simulink model "gm_HFMA_4B_1_5_9_13"  (R2026b)
settings: Solver=FixedStepDiscrete  StopTime=stopTime  FixedStep=1.953125e-06
PreLoadFcn:
  | load('a_luts.mat')
undefined symbols (not defined in the file or in its folder): Ts
libraries: simulink x202, simulink_need_slupdate x99, hdlsllib x91
(part 16 of 20)

== system gm_HFMA_4B_1_5_9_13/Subsystem/HFMA9/crp_temp_shared4 ==
  in0 : Inport  OutDataTypeStr=fixdt(1,18,16,'DataTypeOverride', 'Off')  PortDimensions=1  SampleTime=1.953125e-06
  in1 : Inport  Port=2  OutDataTypeStr=fixdt(1,18,16,'DataTypeOverride', 'Off')  PortDimensions=1  SampleTime=1.953125e-06
  in2 : Inport  Port=3  OutDataTypeStr=fixdt(1,18,16,'DataTypeOverride', 'Off')  PortDimensions=1  SampleTime=1.953125e-06
  in3 : Inport  Port=4  OutDataTypeStr=fixdt(1,18,16,'DataTypeOverride', 'Off')  PortDimensions=1  SampleTime=1.953125e-06
  enb_counter : Inport  Port=5  OutDataTypeStr=fixdt(0,6,0,'DataTypeOverride', 'Off')  PortDimensions=1  SampleTime=1.953125e-06
  Serializer_Subnetwork : Subsystem
  Serializer_Subnetwork1 : Subsystem
  b0_2_const : Constant  Value=0.00121574103832244873046875  OutDataTypeStr=fixdt(1, 18, 26)  SampleTime=1.953125e-06
  b0_2_const1 : Constant  Value=0.00121574103832244873046875  OutDataTypeStr=fixdt(1, 18, 26)  SampleTime=1.953125e-06
  b0_2_const2 : Constant  Value=0.00121574103832244873046875  OutDataTypeStr=fixdt(1, 18, 26)  SampleTime=1.953125e-06
  b1_2 : Product  Inputs=**  OutDataTypeStr=fixdt(1, 36, 0)  SampleTime=1.953125e-06
  b1_2_const{,1..3} (4 alike) : Constant  Value=0.0024314820766448974609375  OutDataTypeStr=fixdt(1, 18, 25)  SampleTime=1.953125e-06
  b2_2_const : Constant  Value=0.00121574103832244873046875  OutDataTypeStr=fixdt(1, 18, 26)  SampleTime=1.953125e-06
  b2_2_const1 : Constant  Value=0.00121574103832244873046875  OutDataTypeStr=fixdt(1, 18, 26)  SampleTime=1.953125e-06
  b2_2_const2 : Constant  Value=0.00121574103832244873046875  OutDataTypeStr=fixdt(1, 18, 26)  SampleTime=1.953125e-06
  counter : Subsystem
  counter_matching_delay : Delay  DelayLength=80  InitialCondition=0  SampleTime=1.953125e-06
  delayMatch : Delay  DelayLength=56  InitialCondition=0  SampleTime=1.953125e-06
  delayMatch{1..13} (13 alike) : Delay  DelayLength=16  InitialCondition=0  SampleTime=1.953125e-06
  delayMatch14 : Delay  DelayLength=24  InitialCondition=0  SampleTime=1.953125e-06
  demux : Demux  Outputs=16
  enb_counter_eq_31 : simulink/Logic and Bit Operations/Compare To Constant  relop===  const=31  OutDataTypeStr=boolean
  enb_counter_ge_16 : simulink/Logic and Bit Operations/Compare To Constant  relop=>=  const=16  OutDataTypeStr=boolean
  enb_counter_ge_16_and_enb_counter_le_31 : Logic  AllPortsSameDT=off  OutDataTypeStr=boolean  SampleTime=1.953125e-06
  enb_counter_le_15 : simulink/Logic and Bit Operations/Compare To Constant  relop=<=  const=15  OutDataTypeStr=boolean
  enb_counter_le_31 : simulink/Logic and Bit Operations/Compare To Constant  relop=<=  const=31  OutDataTypeStr=boolean
  mux : Mux  Inputs=16
  mux1 : Mux  Inputs=16
  na1_1_const : Constant  Value=1.872802734375  OutDataTypeStr=fixdt(1, 18, 16)  SampleTime=1.953125e-06
  na1_1_const1 : Constant  Value=1.872802734375  OutDataTypeStr=fixdt(1, 18, 16)  SampleTime=1.953125e-06
  na1_1_const2 : Constant  Value=1.872802734375  OutDataTypeStr=fixdt(1, 18, 16)  SampleTime=1.953125e-06
  na2_1_const : Constant  Value=-0.87749481201171875  OutDataTypeStr=fixdt(1, 18, 17)  SampleTime=1.953125e-06
  na2_1_const1 : Constant  Value=-0.87749481201171875  OutDataTypeStr=fixdt(1, 18, 17)  SampleTime=1.953125e-06
  na2_1_const2 : Constant  Value=-0.87749481201171875  OutDataTypeStr=fixdt(1, 18, 17)  SampleTime=1.953125e-06
  nequ_dtc{,1..31} (32 alike) : DataTypeConversion  OutDataTypeStr=fixdt(1, 18, 0)  ConvertRealWorld=Stored Integer (SI)  SampleTime=1.953125e-06  SaturateOnIntegerOverflow=off  RndMeth=Floor
  nequ_dtc{32,37,42,47} (4 alike) : DataTypeConversion  OutDataTypeStr=fixdt(1, 36, 41)  ConvertRealWorld=Stored Integer (SI)  SampleTime=1.953125e-06  SaturateOnIntegerOverflow=off  RndMeth=Floor
  nequ_dtc33 : DataTypeConversion  OutDataTypeStr=fixdt(1, 36, 33)  ConvertRealWorld=Stored Integer (SI)  SampleTime=1.953125e-06  SaturateOnIntegerOverflow=off  RndMeth=Floor
  nequ_dtc34 : DataTypeConversion  OutDataTypeStr=fixdt(1, 36, 32)  ConvertRealWorld=Stored Integer (SI)  SampleTime=1.953125e-06  SaturateOnIntegerOverflow=off  RndMeth=Floor
  nequ_dtc{35..36,40..41,45..46} (6 alike) : DataTypeConversion  OutDataTypeStr=fixdt(1, 36, 42)  ConvertRealWorld=Stored Integer (SI)  SampleTime=1.953125e-06  SaturateOnIntegerOverflow=off  RndMeth=Floor
  nequ_dtc38 : DataTypeConversion  OutDataTypeStr=fixdt(1, 36, 33)  ConvertRealWorld=Stored Integer (SI)  SampleTime=1.953125e-06  SaturateOnIntegerOverflow=off  RndMeth=Floor
  nequ_dtc39 : DataTypeConversion  OutDataTypeStr=fixdt(1, 36, 32)  ConvertRealWorld=Stored Integer (SI)  SampleTime=1.953125e-06  SaturateOnIntegerOverflow=off  RndMeth=Floor
  nequ_dtc43 : DataTypeConversion  OutDataTypeStr=fixdt(1, 36, 33)  ConvertRealWorld=Stored Integer (SI)  SampleTime=1.953125e-06  SaturateOnIntegerOverflow=off  RndMeth=Floor
  nequ_dtc44 : DataTypeConversion  OutDataTypeStr=fixdt(1, 36, 32)  ConvertRealWorld=Stored Integer (SI)  SampleTime=1.953125e-06  SaturateOnIntegerOverflow=off  RndMeth=Floor
  tapped_delay : hdlsllib/Discrete/Tapped Delay Enabled Synchronous  vinit=0  samptime=-1  NumDelays=15  DelayOrder=Oldest  includeCurrent=on
  tapped_delay_outunit_delay : simulink_need_slupdate/Unit Delay Enabled  vinit=0.0  tsamp=-1
  out0 : Outport  OutDataTypeStr=fixdt(1,36,41,'DataTypeOverride', 'Off')  PortDimensions=1  SampleTime=1.953125e-06
  out1 : Outport  Port=2  OutDataTypeStr=fixdt(1,36,33,'DataTypeOverride', 'Off')  PortDimensions=1  SampleTime=1.953125e-06
  out2 : Outport  Port=3  OutDataTypeStr=fixdt(1,36,32,'DataTypeOverride', 'Off')  PortDimensions=1  SampleTime=1.953125e-06
  out3 : Outport  Port=4  OutDataTypeStr=fixdt(1,36,42,'DataTypeOverride', 'Off')  PortDimensions=1  SampleTime=1.953125e-06
  out4 : Outport  Port=5  OutDataTypeStr=fixdt(1,36,42,'DataTypeOverride', 'Off')  PortDimensions=1  SampleTime=1.953125e-06
  out5 : Outport  Port=6  OutDataTypeStr=fixdt(1,36,41,'DataTypeOverride', 'Off')  PortDimensions=1  SampleTime=1.953125e-06
  out6 : Outport  Port=7  OutDataTypeStr=fixdt(1,36,33,'DataTypeOverride', 'Off')  PortDimensions=1  SampleTime=1.953125e-06
  out7 : Outport  Port=8  OutDataTypeStr=fixdt(1,36,32,'DataTypeOverride', 'Off')  PortDimensions=1  SampleTime=1.953125e-06
  out8 : Outport  Port=9  OutDataTypeStr=fixdt(1,36,42,'DataTypeOverride', 'Off')  PortDimensions=1  SampleTime=1.953125e-06
  out9 : Outport  Port=10  OutDataTypeStr=fixdt(1,36,42,'DataTypeOverride', 'Off')  PortDimensions=1  SampleTime=1.953125e-06
  out10 : Outport  Port=11  OutDataTypeStr=fixdt(1,36,41,'DataTypeOverride', 'Off')  PortDimensions=1  SampleTime=1.953125e-06
  out11 : Outport  Port=12  OutDataTypeStr=fixdt(1,36,33,'DataTypeOverride', 'Off')  PortDimensions=1  SampleTime=1.953125e-06
  out12 : Outport  Port=13  OutDataTypeStr=fixdt(1,36,32,'DataTypeOverride', 'Off')  PortDimensions=1  SampleTime=1.953125e-06
  out13 : Outport  Port=14  OutDataTypeStr=fixdt(1,36,42,'DataTypeOverride', 'Off')  PortDimensions=1  SampleTime=1.953125e-06
  out14 : Outport  Port=15  OutDataTypeStr=fixdt(1,36,42,'DataTypeOverride', 'Off')  PortDimensions=1  SampleTime=1.953125e-06
  out15 : Outport  Port=16  OutDataTypeStr=fixdt(1,36,41,'DataTypeOverride', 'Off')  PortDimensions=1  SampleTime=1.953125e-06
  wires:
  nequ_dtc25/1 -> delayMatch10/1
  b1_2_const/1 -> nequ_dtc/1
  na1_1_const/1 -> nequ_dtc2/1
  nequ_dtc27/1 -> delayMatch12/1
  na2_1_const/1 -> nequ_dtc1/1
  b0_2_const1/1 -> nequ_dtc9/1
  mux1/1 -> Serializer_Subnetwork1/1(in0)
  b2_2_const/1 -> nequ_dtc3/1
  b1_2_const1/1 -> nequ_dtc5/1
  na1_1_const1/1 -> nequ_dtc7/1
  nequ_dtc15/1 -> mux/16
  b1_2_const2/1 -> nequ_dtc10/1
  b2_2_const1/1 -> nequ_dtc8/1
  b0_2_const/1 -> nequ_dtc4/1
  na2_1_const1/1 -> nequ_dtc6/1
  b1_2_const3/1 -> nequ_dtc15/1
  b2_2_const2/1 -> nequ_dtc13/1
  na2_1_const2/1 -> nequ_dtc11/1
  nequ_dtc17/1 -> delayMatch2/1
  mux/1 -> Serializer_Subnetwork/1(in0)
  b0_2_const2/1 -> nequ_dtc14/1
  na1_1_const2/1 -> nequ_dtc12/1
  delayMatch13/1 -> mux1/13
  in0/1 -> nequ_dtc18/1, nequ_dtc17/1, nequ_dtc16/1
  delayMatch7/1 -> mux1/7
  in1/1 -> nequ_dtc22/1, nequ_dtc21/1, nequ_dtc23/1, nequ_dtc20/1, nequ_dtc19/1
  delayMatch9/1 -> mux1/9
  in2/1 -> nequ_dtc28/1, nequ_dtc27/1, nequ_dtc26/1, nequ_dtc24/1, nequ_dtc25/1
  nequ_dtc18/1 -> delayMatch3/1
  enb_counter/1 -> enb_counter_le_31/1, enb_counter_ge_16/1, enb_counter_le_15/1, enb_counter_eq_31/1
  nequ_dtc36/1 -> out4/1
  nequ_dtc/1 -> mux/1
  nequ_dtc1/1 -> mux/2
  nequ_dtc2/1 -> mux/3
  nequ_dtc6/1 -> mux/7
  nequ_dtc3/1 -> mux/4
  nequ_dtc40/1 -> out8/1
  nequ_dtc4/1 -> mux/5
  nequ_dtc5/1 -> mux/6
  enb_counter_le_31/1 -> enb_counter_ge_16_and_enb_counter_le_31/2
  nequ_dtc7/1 -> mux/8
  nequ_dtc8/1 -> mux/9
  nequ_dtc13/1 -> mux/14
  nequ_dtc9/1 -> mux/10
  nequ_dtc10/1 -> mux/11
  nequ_dtc11/1 -> mux/12
  nequ_dtc12/1 -> mux/13
  nequ_dtc14/1 -> mux/15
  nequ_dtc16/1 -> delayMatch1/1
  in3/1 -> nequ_dtc30/1, nequ_dtc31/1, nequ_dtc29/1
  nequ_dtc23/1 -> delayMatch8/1
  nequ_dtc19/1 -> delayMatch4/1
  nequ_dtc20/1 -> delayMatch5/1
  nequ_dtc21/1 -> delayMatch6/1
  nequ_dtc22/1 -> delayMatch7/1
  enb_counter_le_15/1 -> counter/Enable
  nequ_dtc28/1 -> delayMatch13/1
  nequ_dtc24/1 -> delayMatch9/1
  nequ_dtc26/1 -> delayMatch11/1
  enb_counter_ge_16/1 -> enb_counter_ge_16_and_enb_counter_le_31/1
  delayMatch1/1 -> mux1/1
  delayMatch6/1 -> mux1/6
  delayMatch2/1 -> mux1/2
  delayMatch3/1 -> mux1/3
  delayMatch4/1 -> mux1/4
  delayMatch5/1 -> mux1/5
  delayMatch8/1 -> mux1/8
  counter/1(out0) -> counter_matching_delay/1, Serializer_Subnetwork/2(in1)
  delayMatch10/1 -> mux1/10
  delayMatch11/1 -> mux1/11
  delayMatch12/1 -> mux1/12
  nequ_dtc29/1 -> mux1/14
  nequ_dtc30/1 -> mux1/15
  nequ_dtc31/1 -> mux1/16
  enb_counter_ge_16_and_enb_counter_le_31/1 -> tapped_delay/2
  Serializer_Subnetwork/1(out0) -> delayMatch/1
  counter_matching_delay/1 -> Serializer_Subnetwork1/2(in1)
  delayMatch/1 -> delayMatch14/1
  Serializer_Subnetwork1/1(out0) -> b1_2/2
  delayMatch14/1 -> b1_2/1
  enb_counter_eq_31/1 -> tapped_delay_outunit_delay/2
  b1_2/1 -> tapped_delay/1
  tapped_delay/1 -> tapped_delay_outunit_delay/1
  tapped_delay_outunit_delay/1 -> demux/1
  demux/1 -> nequ_dtc32/1
  demux/2 -> nequ_dtc33/1
  demux/3 -> nequ_dtc34/1
  demux/4 -> nequ_dtc35/1
  demux/5 -> nequ_dtc36/1
  demux/6 -> nequ_dtc37/1
  demux/7 -> nequ_dtc38/1
  demux/8 -> nequ_dtc39/1
  demux/9 -> nequ_dtc40/1
  demux/10 -> nequ_dtc41/1
  demux/11 -> nequ_dtc42/1
  demux/12 -> nequ_dtc43/1
  demux/13 -> nequ_dtc44/1
  demux/14 -> nequ_dtc45/1
  demux/15 -> nequ_dtc46/1
  demux/16 -> nequ_dtc47/1
  nequ_dtc32/1 -> out0/1
  nequ_dtc33/1 -> out1/1
  nequ_dtc34/1 -> out2/1
  nequ_dtc35/1 -> out3/1
  nequ_dtc37/1 -> out5/1
  nequ_dtc38/1 -> out6/1
  nequ_dtc39/1 -> out7/1
  nequ_dtc41/1 -> out9/1
  nequ_dtc42/1 -> out10/1
  nequ_dtc43/1 -> out11/1
  nequ_dtc44/1 -> out12/1
  nequ_dtc45/1 -> out13/1
  nequ_dtc46/1 -> out14/1
  nequ_dtc47/1 -> out15/1

== system gm_HFMA_4B_1_5_9_13/Subsystem/HFMA9/crp_temp_shared5 ==
  in0 : Inport  OutDataTypeStr=fixdt(1,18,16,'DataTypeOverride', 'Off')  PortDimensions=1  SampleTime=1.953125e-06
  in1 : Inport  Port=2  OutDataTypeStr=fixdt(1,18,16,'DataTypeOverride', 'Off')  PortDimensions=1  SampleTime=1.953125e-06
  in2 : Inport  Port=3  OutDataTypeStr=fixdt(1,18,16,'DataTypeOverride', 'Off')  PortDimensions=1  SampleTime=1.953125e-06
  in3 : Inport  Port=4  OutDataTypeStr=fixdt(1,18,16,'DataTypeOverride', 'Off')  PortDimensions=1  SampleTime=1.953125e-06
  enb_counter : Inport  Port=5  OutDataTypeStr=fixdt(0,6,0,'DataTypeOverride', 'Off')  PortDimensions=1  SampleTime=1.953125e-06
  Serializer_Subnetwork : Subsystem
  Serializer_Subnetwork1 : Subsystem
  b0_2_const : Constant  Value=0.00121574103832244873046875  OutDataTypeStr=fixdt(1, 18, 26)  SampleTime=1.953125e-06
  b0_2_const1 : Constant  Value=0.00121574103832244873046875  OutDataTypeStr=fixdt(1, 18, 26)  SampleTime=1.953125e-06
  b0_2_const2 : Constant  Value=0.00121574103832244873046875  OutDataTypeStr=fixdt(1, 18, 26)  SampleTime=1.953125e-06
  b1_2_const : Constant  Value=0.0024314820766448974609375  OutDataTypeStr=fixdt(1, 18, 25)  SampleTime=1.953125e-06
  b1_2_const1 : Constant  Value=0.0024314820766448974609375  OutDataTypeStr=fixdt(1, 18, 25)  SampleTime=1.953125e-06
  b1_2_const2 : Constant  Value=0.0024314820766448974609375  OutDataTypeStr=fixdt(1, 18, 25)  SampleTime=1.953125e-06
  b2_2_const : Constant  Value=0.00121574103832244873046875  OutDataTypeStr=fixdt(1, 18, 26)  SampleTime=1.953125e-06
  b2_2_const1 : Constant  Value=0.00121574103832244873046875  OutDataTypeStr=fixdt(1, 18, 26)  SampleTime=1.953125e-06
  b2_2_const2 : Constant  Value=0.00121574103832244873046875  OutDataTypeStr=fixdt(1, 18, 26)  SampleTime=1.953125e-06
  counter : Subsystem
  counter_matching_delay : Delay  DelayLength=80  InitialCondition=0  SampleTime=1.953125e-06
  delayMatch : Delay  DelayLength=56  InitialCondition=0  SampleTime=1.953125e-06
  delayMatch1 : Delay  DelayLength=24  InitialCondition=0  SampleTime=1.953125e-06
  demux : Demux  Outputs=16
  enb_counter_eq_31 : simulink/Logic and Bit Operations/Compare To Constant  relop===  const=31  OutDataTypeStr=boolean
  enb_counter_ge_16 : simulink/Logic and Bit Operations/Compare To Constant  relop=>=  const=16  OutDataTypeStr=boolean
  enb_counter_ge_16_and_enb_counter_le_31 : Logic  AllPortsSameDT=off  OutDataTypeStr=boolean  SampleTime=1.953125e-06
  enb_counter_le_15 : simulink/Logic and Bit Operations/Compare To Constant  relop=<=  const=15  OutDataTypeStr=boolean
  enb_counter_le_31 : simulink/Logic and Bit Operations/Compare To Constant  relop=<=  const=31  OutDataTypeStr=boolean
  mux : Mux  Inputs=16
  mux1 : Mux  Inputs=16
  na1_1_const : Constant  Value=1.872802734375  OutDataTypeStr=fixdt(1, 18, 16)  SampleTime=1.953125e-06
  na1_1_const1 : Constant  Value=1.872802734375  OutDataTypeStr=fixdt(1, 18, 16)  SampleTime=1.953125e-06
  na1_1_const2 : Constant  Value=1.872802734375  OutDataTypeStr=fixdt(1, 18, 16)  SampleTime=1.953125e-06
  na2_1 : Product  Inputs=**  OutDataTypeStr=fixdt(1, 36, 0)  SampleTime=1.953125e-06
  na2_1_const{,1..3} (4 alike) : Constant  Value=-0.87749481201171875  OutDataTypeStr=fixdt(1, 18, 17)  SampleTime=1.953125e-06
  nequ_dtc{,1..31} (32 alike) : DataTypeConversion  OutDataTypeStr=fixdt(1, 18, 0)  ConvertRealWorld=Stored Integer (SI)  SampleTime=1.953125e-06  SaturateOnIntegerOverflow=off  RndMeth=Floor
  nequ_dtc{32,37,42,47} (4 alike) : DataTypeConversion  OutDataTypeStr=fixdt(1, 36, 33)  ConvertRealWorld=Stored Integer (SI)  SampleTime=1.953125e-06  SaturateOnIntegerOverflow=off  RndMeth=Floor
  nequ_dtc33 : DataTypeConversion  OutDataTypeStr=fixdt(1, 36, 32)  ConvertRealWorld=Stored Integer (SI)  SampleTime=1.953125e-06  SaturateOnIntegerOverflow=off  RndMeth=Floor
  nequ_dtc{34..35,39..40,44..45} (6 alike) : DataTypeConversion  OutDataTypeStr=fixdt(1, 36, 42)  ConvertRealWorld=Stored Integer (SI)  SampleTime=1.953125e-06  SaturateOnIntegerOverflow=off  RndMeth=Floor
  nequ_dtc36 : DataTypeConversion  OutDataTypeStr=fixdt(1, 36, 41)  ConvertRealWorld=Stored Integer (SI)  SampleTime=1.953125e-06  SaturateOnIntegerOverflow=off  RndMeth=Floor
  nequ_dtc38 : DataTypeConversion  OutDataTypeStr=fixdt(1, 36, 32)  ConvertRealWorld=Stored Integer (SI)  SampleTime=1.953125e-06  SaturateOnIntegerOverflow=off  RndMeth=Floor
  nequ_dtc41 : DataTypeConversion  OutDataTypeStr=fixdt(1, 36, 41)  ConvertRealWorld=Stored Integer (SI)  SampleTime=1.953125e-06  SaturateOnIntegerOverflow=off  RndMeth=Floor
  nequ_dtc43 : DataTypeConversion  OutDataTypeStr=fixdt(1, 36, 32)  ConvertRealWorld=Stored Integer (SI)  SampleTime=1.953125e-06  SaturateOnIntegerOverflow=off  RndMeth=Floor
  nequ_dtc46 : DataTypeConversion  OutDataTypeStr=fixdt(1, 36, 41)  ConvertRealWorld=Stored Integer (SI)  SampleTime=1.953125e-06  SaturateOnIntegerOverflow=off  RndMeth=Floor
  tapped_delay : hdlsllib/Discrete/Tapped Delay Enabled Synchronous  vinit=0  samptime=-1  NumDelays=15  DelayOrder=Oldest  includeCurrent=on
  tapped_delay_outunit_delay : simulink_need_slupdate/Unit Delay Enabled  vinit=0.0  tsamp=-1
  out0 : Outport  OutDataTypeStr=fixdt(1,36,33,'DataTypeOverride', 'Off')  PortDimensions=1  SampleTime=1.953125e-06
  out1 : Outport  Port=2  OutDataTypeStr=fixdt(1,36,32,'DataTypeOverride', 'Off')  PortDimensions=1  SampleTime=1.953125e-06
  out2 : Outport  Port=3  OutDataTypeStr=fixdt(1,36,42,'DataTypeOverride', 'Off')  PortDimensions=1  SampleTime=1.953125e-06
  out3 : Outport  Port=4  OutDataTypeStr=fixdt(1,36,42,'DataTypeOverride', 'Off')  PortDimensions=1  SampleTime=1.953125e-06
  out4 : Outport  Port=5  OutDataTypeStr=fixdt(1,36,41,'DataTypeOverride', 'Off')  PortDimensions=1  SampleTime=1.953125e-06
  out5 : Outport  Port=6  OutDataTypeStr=fixdt(1,36,33,'DataTypeOverride', 'Off')  PortDimensions=1  SampleTime=1.953125e-06
  out6 : Outport  Port=7  OutDataTypeStr=fixdt(1,36,32,'DataTypeOverride', 'Off')  PortDimensions=1  SampleTime=1.953125e-06
  out7 : Outport  Port=8  OutDataTypeStr=fixdt(1,36,42,'DataTypeOverride', 'Off')  PortDimensions=1  SampleTime=1.953125e-06
  out8 : Outport  Port=9  OutDataTypeStr=fixdt(1,36,42,'DataTypeOverride', 'Off')  PortDimensions=1  SampleTime=1.953125e-06
  out9 : Outport  Port=10  OutDataTypeStr=fixdt(1,36,41,'DataTypeOverride', 'Off')  PortDimensions=1  SampleTime=1.953125e-06
  out10 : Outport  Port=11  OutDataTypeStr=fixdt(1,36,33,'DataTypeOverride', 'Off')  PortDimensions=1  SampleTime=1.953125e-06
  out11 : Outport  Port=12  OutDataTypeStr=fixdt(1,36,32,'DataTypeOverride', 'Off')  PortDimensions=1  SampleTime=1.953125e-06
  out12 : Outport  Port=13  OutDataTypeStr=fixdt(1,36,42,'DataTypeOverride', 'Off')  PortDimensions=1  SampleTime=1.953125e-06
  out13 : Outport  Port=14  OutDataTypeStr=fixdt(1,36,42,'DataTypeOverride', 'Off')  PortDimensions=1  SampleTime=1.953125e-06
  out14 : Outport  Port=15  OutDataTypeStr=fixdt(1,36,41,'DataTypeOverride', 'Off')  PortDimensions=1  SampleTime=1.953125e-06
  out15 : Outport  Port=16  OutDataTypeStr=fixdt(1,36,33,'DataTypeOverride', 'Off')  PortDimensions=1  SampleTime=1.953125e-06
  wires:
  b0_2_const/1 -> nequ_dtc3/1
  nequ_dtc29/1 -> mux1/14
  na1_1_const/1 -> nequ_dtc1/1
  nequ_dtc25/1 -> mux1/10
  nequ_dtc27/1 -> mux1/12
  na2_1_const/1 -> nequ_dtc/1
  b2_2_const/1 -> nequ_dtc2/1
  demux/8 -> nequ_dtc39/1
  na1_1_const2/1 -> nequ_dtc11/1
  b1_2_const1/1 -> nequ_dtc9/1
  demux/4 -> nequ_dtc35/1
  na2_1_const1/1 -> nequ_dtc5/1
  b2_2_const1/1 -> nequ_dtc7/1
  b0_2_const1/1 -> nequ_dtc8/1
  nequ_dtc31/1 -> mux1/16
  demux/10 -> nequ_dtc41/1
  na2_1_const2/1 -> nequ_dtc10/1
  demux/6 -> nequ_dtc37/1
  b1_2_const/1 -> nequ_dtc4/1
  na1_1_const1/1 -> nequ_dtc6/1
  mux/1 -> Serializer_Subnetwork/1(in0)
  nequ_dtc19/1 -> mux1/4
  b1_2_const2/1 -> nequ_dtc14/1
  b2_2_const2/1 -> nequ_dtc12/1
  b0_2_const2/1 -> nequ_dtc13/1
  nequ_dtc17/1 -> mux1/2
  na2_1_const3/1 -> nequ_dtc15/1
  enb_counter/1 -> enb_counter_le_31/1, enb_counter_ge_16/1, enb_counter_eq_31/1, enb_counter_le_15/1
  nequ_dtc24/1 -> mux1/9
  nequ_dtc20/1 -> mux1/5
  nequ_dtc/1 -> mux/1
  nequ_dtc21/1 -> mux1/6
  nequ_dtc1/1 -> mux/2
  nequ_dtc2/1 -> mux/3
  nequ_dtc3/1 -> mux/4
  nequ_dtc42/1 -> out10/1
  nequ_dtc4/1 -> mux/5
  nequ_dtc5/1 -> mux/6
  nequ_dtc6/1 -> mux/7
  nequ_dtc7/1 -> mux/8
  nequ_dtc8/1 -> mux/9
  Serializer_Subnetwork1/1(out0) -> na2_1/2
  nequ_dtc9/1 -> mux/10
  in2/1 -> nequ_dtc25/1, nequ_dtc26/1, nequ_dtc23/1, nequ_dtc24/1, nequ_dtc27/1
  nequ_dtc14/1 -> mux/15
  nequ_dtc10/1 -> mux/11
  in3/1 -> nequ_dtc31/1, nequ_dtc30/1, nequ_dtc29/1, nequ_dtc28/1
  nequ_dtc11/1 -> mux/12
  in0/1 -> nequ_dtc17/1, nequ_dtc16/1
  nequ_dtc12/1 -> mux/13
  in1/1 -> nequ_dtc21/1, nequ_dtc20/1, nequ_dtc19/1, nequ_dtc18/1, nequ_dtc22/1
  nequ_dtc13/1 -> mux/14
  nequ_dtc15/1 -> mux/16
  enb_counter_le_15/1 -> counter/Enable
  enb_counter_ge_16/1 -> enb_counter_ge_16_and_enb_counter_le_31/1
  enb_counter_le_31/1 -> enb_counter_ge_16_and_enb_counter_le_31/2
  nequ_dtc16/1 -> mux1/1
  nequ_dtc18/1 -> mux1/3
  nequ_dtc22/1 -> mux1/7
  nequ_dtc23/1 -> mux1/8
  counter/1(out0) -> Serializer_Subnetwork/2(in1), counter_matching_delay/1
  nequ_dtc30/1 -> mux1/15
  nequ_dtc26/1 -> mux1/11
  nequ_dtc28/1 -> mux1/13
  enb_counter_ge_16_and_enb_counter_le_31/1 -> tapped_delay/2
  Serializer_Subnetwork/1(out0) -> delayMatch/1
  mux1/1 -> Serializer_Subnetwork1/1(in0)
  counter_matching_delay/1 -> Serializer_Subnetwork1/2(in1)
  delayMatch/1 -> delayMatch1/1
  delayMatch1/1 -> na2_1/1
  enb_counter_eq_31/1 -> tapped_delay_outunit_delay/2
  na2_1/1 -> tapped_delay/1
  tapped_delay/1 -> tapped_delay_outunit_delay/1
  tapped_delay_outunit_delay/1 -> demux/1
  demux/1 -> nequ_dtc32/1
  demux/2 -> nequ_dtc33/1
  demux/3 -> nequ_dtc34/1
  demux/5 -> nequ_dtc36/1
  demux/7 -> nequ_dtc38/1
  demux/9 -> nequ_dtc40/1
  demux/11 -> nequ_dtc42/1
  demux/12 -> nequ_dtc43/1
  demux/13 -> nequ_dtc44/1
  demux/14 -> nequ_dtc45/1
  demux/15 -> nequ_dtc46/1
  demux/16 -> nequ_dtc47/1
  nequ_dtc32/1 -> out0/1
  nequ_dtc33/1 -> out1/1
  nequ_dtc34/1 -> out2/1
  nequ_dtc35/1 -> out3/1
  nequ_dtc36/1 -> out4/1
  nequ_dtc37/1 -> out5/1
  nequ_dtc38/1 -> out6/1
  nequ_dtc39/1 -> out7/1
  nequ_dtc40/1 -> out8/1
  nequ_dtc41/1 -> out9/1
  nequ_dtc43/1 -> out11/1
  nequ_dtc44/1 -> out12/1
  nequ_dtc45/1 -> out13/1
  nequ_dtc46/1 -> out14/1
  nequ_dtc47/1 -> out15/1

== system gm_HFMA_4B_1_5_9_13/Subsystem/HFMA9/crp_temp_shared6 ==
  in0 : Inport  OutDataTypeStr=fixdt(1,18,16,'DataTypeOverride', 'Off')  PortDimensions=1  SampleTime=1.953125e-06
  in1 : Inport  Port=2  OutDataTypeStr=fixdt(1,18,16,'DataTypeOverride', 'Off')  PortDimensions=1  SampleTime=1.953125e-06
  in2 : Inport  Port=3  OutDataTypeStr=fixdt(1,18,16,'DataTypeOverride', 'Off')  PortDimensions=1  SampleTime=1.953125e-06
  in3 : Inport  Port=4  OutDataTypeStr=fixdt(1,18,16,'DataTypeOverride', 'Off')  PortDimensions=1  SampleTime=1.953125e-06
  in4 : Inport  Port=5  OutDataTypeStr=fixdt(1,18,16,'DataTypeOverride', 'Off')  PortDimensions=1  SampleTime=1.953125e-06
  in5 : Inport  Port=6  OutDataTypeStr=fixdt(1,18,16,'DataTypeOverride', 'Off')  PortDimensions=1  SampleTime=1.953125e-06
  in6 : Inport  Port=7  OutDataTypeStr=fixdt(1,18,16,'DataTypeOverride', 'Off')  PortDimensions=1  SampleTime=1.953125e-06
  enb_counter : Inport  Port=8  OutDataTypeStr=fixdt(0,6,0,'DataTypeOverride', 'Off')  PortDimensions=1  SampleTime=1.953125e-06
  Serializer_Subnetwork : Subsystem
  Serializer_Subnetwork1 : Subsystem
  b0_2_const : Constant  Value=0.00121574103832244873046875  OutDataTypeStr=fixdt(1, 18, 26)  SampleTime=1.953125e-06
  b1_2_const : Constant  Value=0.0024314820766448974609375  OutDataTypeStr=fixdt(1, 18, 25)  SampleTime=1.953125e-06
  b2_2_const : Constant  Value=0.00121574103832244873046875  OutDataTypeStr=fixdt(1, 18, 26)  SampleTime=1.953125e-06
  counter : Subsystem
  delayMatch{,1..7,9..12} (12 alike) : Delay  DelayLength=24  InitialCondition=0  SampleTime=1.953125e-06
  delayMatch{8,13..20} (9 alike) : Delay  DelayLength=16  InitialCondition=0  SampleTime=1.953125e-06
  demux : Demux  Outputs=16
  enb_counter_eq_47 : simulink/Logic and Bit Operations/Compare To Constant  relop===  const=47  OutDataTypeStr=boolean
  enb_counter_ge_32 : simulink/Logic and Bit Operations/Compare To Constant  relop=>=  const=32  OutDataTypeStr=boolean
  enb_counter_ge_32_and_enb_counter_le_47 : Logic  AllPortsSameDT=off  OutDataTypeStr=boolean  SampleTime=1.953125e-06
  enb_counter_le_47 : simulink/Logic and Bit Operations/Compare To Constant  relop=<=  const=47  OutDataTypeStr=boolean
  mux : Mux  Inputs=16
  mux1 : Mux  Inputs=16
  na1_1 : Product  Inputs=**  OutDataTypeStr=fixdt(1, 36, 0)  SampleTime=1.953125e-06
  na1_1_const : Constant  Value=1.872802734375  OutDataTypeStr=fixdt(1, 18, 16)  SampleTime=1.953125e-06
  na1_1_const1 : Constant  Value=1.872802734375  OutDataTypeStr=fixdt(1, 18, 16)  SampleTime=1.953125e-06
  na1_2_const : Constant  Value=1.9425048828125  OutDataTypeStr=fixdt(1, 18, 16)  SampleTime=1.953125e-06
  na1_2_const1 : Constant  Value=1.9425048828125  OutDataTypeStr=fixdt(1, 18, 16)  SampleTime=1.953125e-06
  na1_2_const2 : Constant  Value=1.9425048828125  OutDataTypeStr=fixdt(1, 18, 16)  SampleTime=1.953125e-06
  na2_1_const : Constant  Value=-0.87749481201171875  OutDataTypeStr=fixdt(1, 18, 17)  SampleTime=1.953125e-06
  na2_2_const : Constant  Value=-0.94736480712890625  OutDataTypeStr=fixdt(1, 18, 17)  SampleTime=1.953125e-06
  na2_2_const1 : Constant  Value=-0.94736480712890625  OutDataTypeStr=fixdt(1, 18, 17)  SampleTime=1.953125e-06
  na2_2_const2 : Constant  Value=-0.94736480712890625  OutDataTypeStr=fixdt(1, 18, 17)  SampleTime=1.953125e-06
  nequ_dtc{,1..31} (32 alike) : DataTypeConversion  OutDataTypeStr=fixdt(1, 18, 0)  ConvertRealWorld=Stored Integer (SI)  SampleTime=1.953125e-06  SaturateOnIntegerOverflow=off  RndMeth=Floor
  nequ_dtc{32,37,39..40,42..44,46..47} (9 alike) : DataTypeConversion  OutDataTypeStr=fixdt(1, 36, 32)  ConvertRealWorld=Stored Integer (SI)  SampleTime=1.953125e-06  SaturateOnIntegerOverflow=off  RndMeth=Floor
  nequ_dtc33 : DataTypeConversion  OutDataTypeStr=fixdt(1, 36, 42)  ConvertRealWorld=Stored Integer (SI)  SampleTime=1.953125e-06  SaturateOnIntegerOverflow=off  RndMeth=Floor
  nequ_dtc34 : DataTypeConversion  OutDataTypeStr=fixdt(1, 36, 42)  ConvertRealWorld=Stored Integer (SI)  SampleTime=1.953125e-06  SaturateOnIntegerOverflow=off  RndMeth=Floor
  nequ_dtc35 : DataTypeConversion  OutDataTypeStr=fixdt(1, 36, 41)  ConvertRealWorld=Stored Integer (SI)  SampleTime=1.953125e-06  SaturateOnIntegerOverflow=off  RndMeth=Floor
  nequ_dtc{36,38,41,45} (4 alike) : DataTypeConversion  OutDataTypeStr=fixdt(1, 36, 33)  ConvertRealWorld=Stored Integer (SI)  SampleTime=1.953125e-06  SaturateOnIntegerOverflow=off  RndMeth=Floor
  tapped_delay : hdlsllib/Discrete/Tapped Delay Enabled Synchronous  vinit=0  samptime=-1  NumDelays=15  DelayOrder=Oldest  includeCurrent=on
  tapped_delay_outunit_delay : simulink_need_slupdate/Unit Delay Enabled  vinit=0.0  tsamp=-1
  out0 : Outport  OutDataTypeStr=fixdt(1,36,32,'DataTypeOverride', 'Off')  PortDimensions=1  SampleTime=1.953125e-06
  out1 : Outport  Port=2  OutDataTypeStr=fixdt(1,36,42,'DataTypeOverride', 'Off')  PortDimensions=1  SampleTime=1.953125e-06
  out2 : Outport  Port=3  OutDataTypeStr=fixdt(1,36,42,'DataTypeOverride', 'Off')  PortDimensions=1  SampleTime=1.953125e-06
  out3 : Outport  Port=4  OutDataTypeStr=fixdt(1,36,41,'DataTypeOverride', 'Off')  PortDimensions=1  SampleTime=1.953125e-06
  out4 : Outport  Port=5  OutDataTypeStr=fixdt(1,36,33,'DataTypeOverride', 'Off')  PortDimensions=1  SampleTime=1.953125e-06
  out5 : Outport  Port=6  OutDataTypeStr=fixdt(1,36,32,'DataTypeOverride', 'Off')  PortDimensions=1  SampleTime=1.953125e-06
  out6 : Outport  Port=7  OutDataTypeStr=fixdt(1,36,33,'DataTypeOverride', 'Off')  PortDimensions=1  SampleTime=1.953125e-06
  out7 : Outport  Port=8  OutDataTypeStr=fixdt(1,36,32,'DataTypeOverride', 'Off')  PortDimensions=1  SampleTime=1.953125e-06
  out8 : Outport  Port=9  OutDataTypeStr=fixdt(1,36,32,'DataTypeOverride', 'Off')  PortDimensions=1  SampleTime=1.953125e-06
  out9 : Outport  Port=10  OutDataTypeStr=fixdt(1,36,33,'DataTypeOverride', 'Off')  PortDimensions=1  SampleTime=1.953125e-06
  out10 : Outport  Port=11  OutDataTypeStr=fixdt(1,36,32,'DataTypeOverride', 'Off')  PortDimensions=1  SampleTime=1.953125e-06
  out11 : Outport  Port=12  OutDataTypeStr=fixdt(1,36,32,'DataTypeOverride', 'Off')  PortDimensions=1  SampleTime=1.953125e-06
  out12 : Outport  Port=13  OutDataTypeStr=fixdt(1,36,32,'DataTypeOverride', 'Off')  PortDimensions=1  SampleTime=1.953125e-06
  out13 : Outport  Port=14  OutDataTypeStr=fixdt(1,36,33,'DataTypeOverride', 'Off')  PortDimensions=1  SampleTime=1.953125e-06
  out14 : Outport  Port=15  OutDataTypeStr=fixdt(1,36,32,'DataTypeOverride', 'Off')  PortDimensions=1  SampleTime=1.953125e-06
  out15 : Outport  Port=16  OutDataTypeStr=fixdt(1,36,32,'DataTypeOverride', 'Off')  PortDimensions=1  SampleTime=1.953125e-06
  wires:
  na1_1_const/1 -> nequ_dtc/1
  demux/3 -> nequ_dtc34/1
  b0_2_const/1 -> nequ_dtc2/1
  demux/15 -> nequ_dtc46/1
  na2_1_const/1 -> nequ_dtc4/1
  demux/5 -> nequ_dtc36/1
  b2_2_const/1 -> nequ_dtc1/1
  b1_2_const/1 -> nequ_dtc3/1
  na1_1_const1/1 -> nequ_dtc5/1
  nequ_dtc20/1 -> delayMatch17/1
  na1_2_const2/1 -> nequ_dtc14/1
  na1_2_const1/1 -> nequ_dtc10/1
  na1_2_const/1 -> nequ_dtc7/1
  nequ_dtc18/1 -> delayMatch15/1
  na2_2_const2/1 -> nequ_dtc13/1
  na2_2_const1/1 -> nequ_dtc9/1
  na2_2_const/1 -> nequ_dtc6/1
  in0/1 -> nequ_dtc16/1
  nequ_dtc12/1 -> mux/13
  in6/1 -> nequ_dtc15/1
  nequ_dtc16/1 -> delayMatch13/1
  in2/1 -> nequ_dtc23/1, nequ_dtc22/1, nequ_dtc8/1
  nequ_dtc13/1 -> delayMatch11/1
  in1/1 -> nequ_dtc21/1, nequ_dtc20/1, nequ_dtc19/1, nequ_dtc18/1, nequ_dtc17/1
  in3/1 -> nequ_dtc31/1, nequ_dtc29/1, nequ_dtc27/1, nequ_dtc30/1, nequ_dtc24/1
  enb_counter/1 -> enb_counter_eq_47/1, enb_counter_le_47/1, enb_counter_ge_32/1
  nequ_dtc/1 -> delayMatch/1
  nequ_dtc1/1 -> delayMatch1/1
  enb_counter_le_47/1 -> enb_counter_ge_32_and_enb_counter_le_47/2
  nequ_dtc6/1 -> delayMatch6/1
  nequ_dtc2/1 -> delayMatch2/1
  nequ_dtc3/1 -> delayMatch3/1
  nequ_dtc4/1 -> delayMatch4/1
  nequ_dtc5/1 -> delayMatch5/1
  nequ_dtc11/1 -> mux/12
  nequ_dtc7/1 -> delayMatch7/1
  nequ_dtc8/1 -> delayMatch8/1
  nequ_dtc9/1 -> delayMatch9/1
  nequ_dtc10/1 -> delayMatch10/1
  nequ_dtc14/1 -> delayMatch12/1
  nequ_dtc21/1 -> delayMatch18/1
  nequ_dtc17/1 -> delayMatch14/1
  in4/1 -> nequ_dtc26/1, nequ_dtc25/1, nequ_dtc12/1, nequ_dtc11/1
  nequ_dtc19/1 -> delayMatch16/1
  nequ_dtc22/1 -> delayMatch19/1
  nequ_dtc23/1 -> delayMatch20/1
  in5/1 -> nequ_dtc28/1
  enb_counter_ge_32/1 -> enb_counter_ge_32_and_enb_counter_le_47/1
  delayMatch4/1 -> mux/5
  delayMatch/1 -> mux/1
  delayMatch5/1 -> mux/6
  delayMatch1/1 -> mux/2
  delayMatch2/1 -> mux/3
  delayMatch3/1 -> mux/4
  delayMatch10/1 -> mux/11
  delayMatch6/1 -> mux/7
  delayMatch7/1 -> mux/8
  delayMatch8/1 -> mux/9
  delayMatch9/1 -> mux/10
  delayMatch15/1 -> mux1/3
  delayMatch11/1 -> mux/14
  delayMatch12/1 -> mux/15
  nequ_dtc15/1 -> mux/16
  delayMatch13/1 -> mux1/1
  delayMatch14/1 -> mux1/2
  delayMatch16/1 -> mux1/4
  delayMatch17/1 -> mux1/5
  delayMatch18/1 -> mux1/6
  delayMatch19/1 -> mux1/7
  delayMatch20/1 -> mux1/8
  nequ_dtc24/1 -> mux1/9
  nequ_dtc25/1 -> mux1/10
  nequ_dtc26/1 -> mux1/11
  nequ_dtc27/1 -> mux1/12
  nequ_dtc28/1 -> mux1/13
  nequ_dtc29/1 -> mux1/14
  nequ_dtc30/1 -> mux1/15
  nequ_dtc31/1 -> mux1/16
  enb_counter_ge_32_and_enb_counter_le_47/1 -> counter/Enable, tapped_delay/2
  mux/1 -> Serializer_Subnetwork/1(in0)
  mux1/1 -> Serializer_Subnetwork1/1(in0)
  counter/1(out0) -> Serializer_Subnetwork1/2(in1), Serializer_Subnetwork/2(in1)
  Serializer_Subnetwork/1(out0) -> na1_1/1
  Serializer_Subnetwork1/1(out0) -> na1_1/2
  na1_1/1 -> tapped_delay/1
  enb_counter_eq_47/1 -> tapped_delay_outunit_delay/2
  tapped_delay/1 -> tapped_delay_outunit_delay/1
  tapped_delay_outunit_delay/1 -> demux/1
  demux/1 -> nequ_dtc32/1
  demux/2 -> nequ_dtc33/1
  demux/4 -> nequ_dtc35/1
  demux/6 -> nequ_dtc37/1
  demux/7 -> nequ_dtc38/1
  demux/8 -> nequ_dtc39/1
  demux/9 -> nequ_dtc40/1
  demux/10 -> nequ_dtc41/1
  demux/11 -> nequ_dtc42/1
  demux/12 -> nequ_dtc43/1
  demux/13 -> nequ_dtc44/1
  demux/14 -> nequ_dtc45/1
  demux/16 -> nequ_dtc47/1
  nequ_dtc32/1 -> out0/1
  nequ_dtc33/1 -> out1/1
  nequ_dtc34/1 -> out2/1
  nequ_dtc35/1 -> out3/1
  nequ_dtc36/1 -> out4/1
  nequ_dtc37/1 -> out5/1
  nequ_dtc38/1 -> out6/1
  nequ_dtc39/1 -> out7/1
  nequ_dtc40/1 -> out8/1
  nequ_dtc41/1 -> out9/1
  nequ_dtc42/1 -> out10/1
  nequ_dtc43/1 -> out11/1
  nequ_dtc44/1 -> out12/1
  nequ_dtc45/1 -> out13/1
  nequ_dtc46/1 -> out14/1
  nequ_dtc47/1 -> out15/1

== system gm_HFMA_4B_1_5_9_13/Subsystem/HFMA9/crp_temp_shared7 ==
  in0 : Inport  OutDataTypeStr=fixdt(1,32,28,'DataTypeOverride', 'Off')  PortDimensions=1  SampleTime=1.953125e-06
  in1 : Inport  Port=2  OutDataTypeStr=fixdt(1,32,28,'DataTypeOverride', 'Off')  PortDimensions=1  SampleTime=1.953125e-06
  enb_counter : Inport  Port=3  OutDataTypeStr=fixdt(0,6,0,'DataTypeOverride', 'Off')  PortDimensions=1  SampleTime=1.953125e-06
  Product1 : Product  Inputs=**  OutDataTypeStr=fixdt(1, 64, 56)  SampleTime=1.953125e-06
  Serializer_Subnetwork : Subsystem
  Serializer_Subnetwork1 : Subsystem
  counter : Subsystem
  demux : Demux  Outputs=2
  enb_counter_eq_55 : simulink/Logic and Bit Operations/Compare To Constant  relop===  const=55  OutDataTypeStr=boolean
  enb_counter_ge_54 : simulink/Logic and Bit Operations/Compare To Constant  relop=>=  const=54  OutDataTypeStr=boolean
  enb_counter_ge_54_and_enb_counter_le_55 : Logic  AllPortsSameDT=off  OutDataTypeStr=boolean  SampleTime=1.953125e-06
  enb_counter_le_55 : simulink/Logic and Bit Operations/Compare To Constant  relop=<=  const=55  OutDataTypeStr=boolean
  mux : Mux  Inputs=2
  mux1 : Mux  Inputs=2
  tapped_delay : hdlsllib/Discrete/Tapped Delay Enabled Synchronous  vinit=0  samptime=-1  NumDelays=1  DelayOrder=Oldest  includeCurrent=on
  tapped_delay_outunit_delay : simulink_need_slupdate/Unit Delay Enabled  vinit=0.0  tsamp=-1
  out0 : Outport  OutDataTypeStr=fixdt(1,64,56,'DataTypeOverride', 'Off')  PortDimensions=1  SampleTime=1.953125e-06
  out1 : Outport  Port=2  OutDataTypeStr=fixdt(1,64,56,'DataTypeOverride', 'Off')  PortDimensions=1  SampleTime=1.953125e-06
  wires:
  in1/1 -> mux1/2, mux/2
  in0/1 -> mux1/1, mux/1
  enb_counter/1 -> enb_counter_le_55/1, enb_counter_eq_55/1, enb_counter_ge_54/1
  enb_counter_ge_54/1 -> enb_counter_ge_54_and_enb_counter_le_55/1
  enb_counter_ge_54_and_enb_counter_le_55/1 -> counter/Enable, tapped_delay/2
  enb_counter_le_55/1 -> enb_counter_ge_54_and_enb_counter_le_55/2
  mux1/1 -> Serializer_Subnetwork1/1(in0)
  mux/1 -> Serializer_Subnetwork/1(in0)
  counter/1(out0) -> Serializer_Subnetwork/2(in1), Serializer_Subnetwork1/2(in1)
  Serializer_Subnetwork/1(out0) -> Product1/1
  Serializer_Subnetwork1/1(out0) -> Product1/2
  Product1/1 -> tapped_delay/1
  enb_counter_eq_55/1 -> tapped_delay_outunit_delay/2
  tapped_delay/1 -> tapped_delay_outunit_delay/1
  tapped_delay_outunit_delay/1 -> demux/1
  demux/1 -> out0/1
  demux/2 -> out1/1

== system gm_HFMA_4B_1_5_9_13/Subsystem/HFMA9/crp_temp_shared8 ==
  in0 : Inport  OutDataTypeStr=fixdt(1,18,16,'DataTypeOverride', 'Off')  PortDimensions=1  SampleTime=1.953125e-06
  in1 : Inport  Port=2  OutDataTypeStr=fixdt(1,18,16,'DataTypeOverride', 'Off')  PortDimensions=1  SampleTime=1.953125e-06
  in2 : Inport  Port=3  OutDataTypeStr=fixdt(1,18,16,'DataTypeOverride', 'Off')  PortDimensions=1  SampleTime=1.953125e-06
  in3 : Inport  Port=4  OutDataTypeStr=fixdt(1,18,16,'DataTypeOverride', 'Off')  PortDimensions=1  SampleTime=1.953125e-06
  in4 : Inport  Port=5  OutDataTypeStr=fixdt(1,18,16,'DataTypeOverride', 'Off')  PortDimensions=1  SampleTime=1.953125e-06
  in5 : Inport  Port=6  OutDataTypeStr=fixdt(1,18,16,'DataTypeOverride', 'Off')  PortDimensions=1  SampleTime=1.953125e-06
  in6 : Inport  Port=7  OutDataTypeStr=fixdt(1,18,16,'DataTypeOverride', 'Off')  PortDimensions=1  SampleTime=1.953125e-06
  enb_counter : Inport  Port=8  OutDataTypeStr=fixdt(0,6,0,'DataTypeOverride', 'Off')  PortDimensions=1  SampleTime=1.953125e-06
  Product : Product  Inputs=**  OutDataTypeStr=fixdt(1, 36, 0)  SampleTime=1.953125e-06
  Serializer_Subnetwork : Subsystem
  Serializer_Subnetwork1 : Subsystem
  counter : Subsystem
  delayMatch : Delay  DelayLength=8  InitialCondition=0  SampleTime=1.953125e-06
  delayMatch{1,4,7,11,14,16..30} (20 alike) : Delay  DelayLength=16  InitialCondition=0  SampleTime=1.953125e-06
  delayMatch{2..3,5..6,8..10,12..13,15} (10 alike) : Delay  DelayLength=24  InitialCondition=0  SampleTime=1.953125e-06
  demux : Demux  Outputs=16
  enb_counter_eq_63 : simulink/Logic and Bit Operations/Compare To Constant  relop===  const=63  OutDataTypeStr=boolean
  enb_counter_ge_48 : simulink/Logic and Bit Operations/Compare To Constant  relop=>=  const=48  OutDataTypeStr=boolean
  mux : Mux  Inputs=16
  mux1 : Mux  Inputs=16
  na1_2_const{,1..3} (4 alike) : Constant  Value=1.9425048828125  OutDataTypeStr=fixdt(1, 18, 16)  SampleTime=1.953125e-06
  na2_2_const{,1..4} (5 alike) : Constant  Value=-0.94736480712890625  OutDataTypeStr=fixdt(1, 18, 17)  SampleTime=1.953125e-06
  nequ_dtc{,1..31} (32 alike) : DataTypeConversion  OutDataTypeStr=fixdt(1, 18, 0)  ConvertRealWorld=Stored Integer (SI)  SampleTime=1.953125e-06  SaturateOnIntegerOverflow=off  RndMeth=Floor
  nequ_dtc{32,34..35,37..38,40..43,45..46} (11 alike) : DataTypeConversion  OutDataTypeStr=fixdt(1, 36, 32)  ConvertRealWorld=Stored Integer (SI)  SampleTime=1.953125e-06  SaturateOnIntegerOverflow=off  RndMeth=Floor
  nequ_dtc{33,36,39,44,47} (5 alike) : DataTypeConversion  OutDataTypeStr=fixdt(1, 36, 33)  ConvertRealWorld=Stored Integer (SI)  SampleTime=1.953125e-06  SaturateOnIntegerOverflow=off  RndMeth=Floor
  tapped_delay : hdlsllib/Discrete/Tapped Delay Enabled Synchronous  vinit=0  samptime=-1  NumDelays=15  DelayOrder=Oldest  includeCurrent=on
  tapped_delay_outunit_delay : simulink_need_slupdate/Unit Delay Enabled  vinit=0.0  tsamp=-1
  out0 : Outport  OutDataTypeStr=fixdt(1,36,32,'DataTypeOverride', 'Off')  PortDimensions=1  SampleTime=1.953125e-06
  out1 : Outport  Port=2  OutDataTypeStr=fixdt(1,36,33,'DataTypeOverride', 'Off')  PortDimensions=1  SampleTime=1.953125e-06
  out2 : Outport  Port=3  OutDataTypeStr=fixdt(1,36,32,'DataTypeOverride', 'Off')  PortDimensions=1  SampleTime=1.953125e-06
  out3 : Outport  Port=4  OutDataTypeStr=fixdt(1,36,32,'DataTypeOverride', 'Off')  PortDimensions=1  SampleTime=1.953125e-06
  out4 : Outport  Port=5  OutDataTypeStr=fixdt(1,36,33,'DataTypeOverride', 'Off')  PortDimensions=1  SampleTime=1.953125e-06
  out5 : Outport  Port=6  OutDataTypeStr=fixdt(1,36,32,'DataTypeOverride', 'Off')  PortDimensions=1  SampleTime=1.953125e-06
  out6 : Outport  Port=7  OutDataTypeStr=fixdt(1,36,32,'DataTypeOverride', 'Off')  PortDimensions=1  SampleTime=1.953125e-06
  out7 : Outport  Port=8  OutDataTypeStr=fixdt(1,36,33,'DataTypeOverride', 'Off')  PortDimensions=1  SampleTime=1.953125e-06
  out8 : Outport  Port=9  OutDataTypeStr=fixdt(1,36,32,'DataTypeOverride', 'Off')  PortDimensions=1  SampleTime=1.953125e-06
  out9 : Outport  Port=10  OutDataTypeStr=fixdt(1,36,32,'DataTypeOverride', 'Off')  PortDimensions=1  SampleTime=1.953125e-06
  out10 : Outport  Port=11  OutDataTypeStr=fixdt(1,36,32,'DataTypeOverride', 'Off')  PortDimensions=1  SampleTime=1.953125e-06
  out11 : Outport  Port=12  OutDataTypeStr=fixdt(1,36,32,'DataTypeOverride', 'Off')  PortDimensions=1  SampleTime=1.953125e-06
  out12 : Outport  Port=13  OutDataTypeStr=fixdt(1,36,33,'DataTypeOverride', 'Off')  PortDimensions=1  SampleTime=1.953125e-06
  out13 : Outport  Port=14  OutDataTypeStr=fixdt(1,36,32,'DataTypeOverride', 'Off')  PortDimensions=1  SampleTime=1.953125e-06
  out14 : Outport  Port=15  OutDataTypeStr=fixdt(1,36,32,'DataTypeOverride', 'Off')  PortDimensions=1  SampleTime=1.953125e-06
  out15 : Outport  Port=16  OutDataTypeStr=fixdt(1,36,33,'DataTypeOverride', 'Off')  PortDimensions=1  SampleTime=1.953125e-06
  wires:
  delayMatch9/1 -> mux/9
  nequ_dtc10/1 -> delayMatch/1
  in5/1 -> nequ_dtc10/1
  na1_2_const/1 -> nequ_dtc2/1
  na1_2_const1/1 -> nequ_dtc5/1
  na1_2_const2/1 -> nequ_dtc8/1
  na2_2_const/1 -> nequ_dtc1/1
  na2_2_const1/1 -> nequ_dtc4/1
  na2_2_const2/1 -> nequ_dtc7/1
  nequ_dtc21/1 -> delayMatch21/1
  in0/1 -> nequ_dtc18/1, nequ_dtc17/1, nequ_dtc3/1, nequ_dtc/1
  na2_2_const4/1 -> nequ_dtc15/1
  na2_2_const3/1 -> nequ_dtc12/1
  na1_2_const3/1 -> nequ_dtc13/1
  in3/1 -> nequ_dtc20/1, nequ_dtc6/1, nequ_dtc21/1
  in2/1 -> nequ_dtc27/1, nequ_dtc24/1, nequ_dtc26/1, nequ_dtc23/1, nequ_dtc22/1, nequ_dtc25/1, nequ_dtc19/1
  in6/1 -> nequ_dtc28/1, nequ_dtc11/1, nequ_dtc14/1, nequ_dtc29/1
  nequ_dtc22/1 -> delayMatch22/1
  nequ_dtc18/1 -> delayMatch18/1
  in1/1 -> nequ_dtc30/1, nequ_dtc16/1
  nequ_dtc/1 -> delayMatch1/1
  nequ_dtc1/1 -> delayMatch2/1
  nequ_dtc2/1 -> delayMatch3/1
  nequ_dtc7/1 -> delayMatch8/1
  nequ_dtc3/1 -> delayMatch4/1
  nequ_dtc4/1 -> delayMatch5/1
  nequ_dtc5/1 -> delayMatch6/1
  nequ_dtc6/1 -> delayMatch7/1
  nequ_dtc12/1 -> delayMatch12/1
  delayMatch11/1 -> mux/12
  delayMatch7/1 -> mux/7
  nequ_dtc8/1 -> delayMatch9/1
  delayMatch/1 -> delayMatch10/1
  delayMatch8/1 -> mux/8
  nequ_dtc11/1 -> delayMatch11/1
  nequ_dtc13/1 -> delayMatch13/1
  nequ_dtc14/1 -> delayMatch14/1
  nequ_dtc15/1 -> delayMatch15/1
  delayMatch17/1 -> mux1/2
  nequ_dtc16/1 -> delayMatch16/1
  nequ_dtc17/1 -> delayMatch17/1
  nequ_dtc19/1 -> delayMatch19/1
  nequ_dtc20/1 -> delayMatch20/1
  nequ_dtc39/1 -> out7/1
  in4/1 -> nequ_dtc31/1, nequ_dtc9/1
  nequ_dtc27/1 -> delayMatch27/1
  nequ_dtc23/1 -> delayMatch23/1
  nequ_dtc28/1 -> delayMatch28/1
  nequ_dtc24/1 -> delayMatch24/1
  nequ_dtc25/1 -> delayMatch25/1
  nequ_dtc26/1 -> delayMatch26/1
  delayMatch5/1 -> mux/5
  delayMatch1/1 -> mux/1
  nequ_dtc29/1 -> delayMatch29/1
  delayMatch4/1 -> mux/4
  nequ_dtc30/1 -> delayMatch30/1
  delayMatch26/1 -> mux1/11
  enb_counter/1 -> enb_counter_eq_63/1, enb_counter_ge_48/1
  delayMatch6/1 -> mux/6
  delayMatch2/1 -> mux/2
  delayMatch3/1 -> mux/3
  delayMatch10/1 -> mux/11
  nequ_dtc9/1 -> mux/10
  delayMatch12/1 -> mux/13
  delayMatch13/1 -> mux/14
  nequ_dtc38/1 -> out6/1
  delayMatch14/1 -> mux/15
  delayMatch15/1 -> mux/16
  delayMatch16/1 -> mux1/1
  delayMatch18/1 -> mux1/3
  delayMatch19/1 -> mux1/4
  delayMatch20/1 -> mux1/5
  delayMatch21/1 -> mux1/6
  delayMatch22/1 -> mux1/7
  nequ_dtc45/1 -> out13/1
  delayMatch23/1 -> mux1/8
  nequ_dtc44/1 -> out12/1
  delayMatch24/1 -> mux1/9
  delayMatch25/1 -> mux1/10
  delayMatch27/1 -> mux1/12
  delayMatch28/1 -> mux1/13
  delayMatch29/1 -> mux1/14
  delayMatch30/1 -> mux1/15
  nequ_dtc31/1 -> mux1/16
  enb_counter_ge_48/1 -> tapped_delay/2, counter/Enable
  mux/1 -> Serializer_Subnetwork/1(in0)
  mux1/1 -> Serializer_Subnetwork1/1(in0)
  counter/1(out0) -> Serializer_Subnetwork1/2(in1), Serializer_Subnetwork/2(in1)
  Serializer_Subnetwork/1(out0) -> Product/1
  Serializer_Subnetwork1/1(out0) -> Product/2
  Product/1 -> tapped_delay/1
  enb_counter_eq_63/1 -> tapped_delay_outunit_delay/2
  tapped_delay/1 -> tapped_delay_outunit_delay/1
  tapped_delay_outunit_delay/1 -> demux/1
  demux/1 -> nequ_dtc32/1
  demux/2 -> nequ_dtc33/1
  demux/3 -> nequ_dtc34/1
  demux/4 -> nequ_dtc35/1
  demux/5 -> nequ_dtc36/1
  demux/6 -> nequ_dtc37/1
  demux/7 -> nequ_dtc38/1
  demux/8 -> nequ_dtc39/1
  demux/9 -> nequ_dtc40/1
  demux/10 -> nequ_dtc41/1
  demux/11 -> nequ_dtc42/1
  demux/12 -> nequ_dtc43/1
  demux/13 -> nequ_dtc44/1
  demux/14 -> nequ_dtc45/1
  demux/15 -> nequ_dtc46/1
  demux/16 -> nequ_dtc47/1
  nequ_dtc32/1 -> out0/1
  nequ_dtc34/1 -> out2/1
  nequ_dtc35/1 -> out3/1
  nequ_dtc47/1 -> out15/1
  nequ_dtc41/1 -> out9/1
  nequ_dtc36/1 -> out4/1
  nequ_dtc40/1 -> out8/1
  nequ_dtc43/1 -> out11/1
  nequ_dtc46/1 -> out14/1
  nequ_dtc33/1 -> out1/1
  nequ_dtc42/1 -> out10/1
  nequ_dtc37/1 -> out5/1

== system gm_HFMA_4B_1_5_9_13/Subsystem/HFMA9/crp_temp_shared9 ==
  in0 : Inport  OutDataTypeStr=fixdt(1,18,16,'DataTypeOverride', 'Off')  PortDimensions=1  SampleTime=1.953125e-06
  in1 : Inport  Port=2  OutDataTypeStr=fixdt(1,18,16,'DataTypeOverride', 'Off')  PortDimensions=1  SampleTime=1.953125e-06
  enb_counter : Inport  Port=3  OutDataTypeStr=fixdt(0,6,0,'DataTypeOverride', 'Off')  PortDimensions=1  SampleTime=1.953125e-06
  Serializer_Subnetwork : Subsystem
  Serializer_Subnetwork1 : Subsystem
  counter : Subsystem
  delayMatch : Delay  DelayLength=24  InitialCondition=0  SampleTime=1.953125e-06
  delayMatch1 : Delay  DelayLength=16  InitialCondition=0  SampleTime=1.953125e-06
  demux : Demux  Outputs=2
  enb_counter_eq_49 : simulink/Logic and Bit Operations/Compare To Constant  relop===  const=49  OutDataTypeStr=boolean
  enb_counter_ge_48 : simulink/Logic and Bit Operations/Compare To Constant  relop=>=  const=48  OutDataTypeStr=boolean
  enb_counter_ge_48_and_enb_counter_le_49 : Logic  AllPortsSameDT=off  OutDataTypeStr=boolean  SampleTime=1.953125e-06
  enb_counter_le_49 : simulink/Logic and Bit Operations/Compare To Constant  relop=<=  const=49  OutDataTypeStr=boolean
  mux : Mux  Inputs=2
  mux1 : Mux  Inputs=2
  na1_2 : Product  Inputs=**  OutDataTypeStr=fixdt(1, 36, 32)  SampleTime=1.953125e-06
  na1_2_const : Constant  Value=1.9425048828125  OutDataTypeStr=fixdt(1, 18, 16)  SampleTime=1.953125e-06
  tapped_delay : hdlsllib/Discrete/Tapped Delay Enabled Synchronous  vinit=0  samptime=-1  NumDelays=1  DelayOrder=Oldest  includeCurrent=on
  tapped_delay_outunit_delay : simulink_need_slupdate/Unit Delay Enabled  vinit=0.0  tsamp=-1
  out0 : Outport  OutDataTypeStr=fixdt(1,36,32,'DataTypeOverride', 'Off')  PortDimensions=1  SampleTime=1.953125e-06
  out1 : Outport  Port=2  OutDataTypeStr=fixdt(1,36,32,'DataTypeOverride', 'Off')  PortDimensions=1  SampleTime=1.953125e-06
  wires:
  in0/1 -> mux1/1, mux/2
  in1/1 -> delayMatch1/1
  enb_counter/1 -> enb_counter_eq_49/1, enb_counter_le_49/1, enb_counter_ge_48/1
  demux/2 -> out1/1
  na1_2_const/1 -> delayMatch/1
  enb_counter_ge_48/1 -> enb_counter_ge_48_and_enb_counter_le_49/1
  delayMatch/1 -> mux/1
  enb_counter_le_49/1 -> enb_counter_ge_48_and_enb_counter_le_49/2
  enb_counter_ge_48_and_enb_counter_le_49/1 -> tapped_delay/2, counter/Enable
  delayMatch1/1 -> mux1/2
  na1_2/1 -> tapped_delay/1
  mux1/1 -> Serializer_Subnetwork1/1(in0)
  mux/1 -> Serializer_Subnetwork/1(in0)
  counter/1(out0) -> Serializer_Subnetwork1/2(in1), Serializer_Subnetwork/2(in1)
  Serializer_Subnetwork/1(out0) -> na1_2/1
  Serializer_Subnetwork1/1(out0) -> na1_2/2
  enb_counter_eq_49/1 -> tapped_delay_outunit_delay/2
  tapped_delay/1 -> tapped_delay_outunit_delay/1
  tapped_delay_outunit_delay/1 -> demux/1
  demux/1 -> out0/1

== system gm_HFMA_4B_1_5_9_13/Subsystem/crp_temp_shared/Serializer_Subnetwork ==
  in0 : Inport  OutDataTypeStr=fixdt(1,19,0,'DataTypeOverride', 'Off')  PortDimensions=[16]  SampleTime=1.953125e-06
  in1 : Inport  Port=2  OutDataTypeStr=fixdt(0,4,0,'DataTypeOverride', 'Off')  PortDimensions=1  SampleTime=1.953125e-06
  ratechange_splitcomp : Demux  Outputs=16
  splitcomp_multiport : MultiPortSwitch  DataPortOrder=Zero-based contiguous  Inputs=16  DiagnosticForDefault=None  zeroidx=on  OutDataTypeStr=fixdt(1, 19, 0)  SampleTime=1.953125e-06  SaturateOnIntegerOverflow=off  InputSameDT=off
  out0 : Outport  OutDataTypeStr=fixdt(1,19,0,'DataTypeOverride', 'Off')  PortDimensions=1  SampleTime=1.953125e-06
  wires:
  splitcomp_multiport/1 -> out0/1
  ratechange_splitcomp/14 -> splitcomp_multiport/15
  in0/1 -> ratechange_splitcomp/1
  in1/1 -> splitcomp_multiport/1
  ratechange_splitcomp/10 -> splitcomp_multiport/11
  ratechange_splitcomp/2 -> splitcomp_multiport/3
  ratechange_splitcomp/6 -> splitcomp_multiport/7
  ratechange_splitcomp/9 -> splitcomp_multiport/10
  ratechange_splitcomp/1 -> splitcomp_multiport/2
  ratechange_splitcomp/5 -> splitcomp_multiport/6
  ratechange_splitcomp/8 -> splitcomp_multiport/9
  ratechange_splitcomp/4 -> splitcomp_multiport/5
  ratechange_splitcomp/7 -> splitcomp_multiport/8
  ratechange_splitcomp/3 -> splitcomp_multiport/4
  ratechange_splitcomp/15 -> splitcomp_multiport/16
  ratechange_splitcomp/11 -> splitcomp_multiport/12
  ratechange_splitcomp/16 -> splitcomp_multiport/17
  ratechange_splitcomp/12 -> splitcomp_multiport/13
  ratechange_splitcomp/13 -> splitcomp_multiport/14

== system gm_HFMA_4B_1_5_9_13/Subsystem/crp_temp_shared/Serializer_Subnetwork1 ==
  in0 : Inport  OutDataTypeStr=fixdt(1,17,0,'DataTypeOverride', 'Off')  PortDimensions=[16]  SampleTime=1.953125e-06
  in1 : Inport  Port=2  OutDataTypeStr=fixdt(0,4,0,'DataTypeOverride', 'Off')  PortDimensions=1  SampleTime=1.953125e-06
  ratechange_splitcomp : Demux  Outputs=16
  splitcomp_multiport : MultiPortSwitch  DataPortOrder=Zero-based contiguous  Inputs=16  DiagnosticForDefault=None  zeroidx=on  OutDataTypeStr=fixdt(1, 17, 0)  SampleTime=1.953125e-06  SaturateOnIntegerOverflow=off  InputSameDT=off
  out0 : Outport  OutDataTypeStr=fixdt(1,17,0,'DataTypeOverride', 'Off')  PortDimensions=1  SampleTime=1.953125e-06
  wires:
  in1/1 -> splitcomp_multiport/1
  in0/1 -> ratechange_splitcomp/1
  splitcomp_multiport/1 -> out0/1
  ratechange_splitcomp/14 -> splitcomp_multiport/15
  ratechange_splitcomp/10 -> splitcomp_multiport/11
  ratechange_splitcomp/2 -> splitcomp_multiport/3
  ratechange_splitcomp/6 -> splitcomp_multiport/7
  ratechange_splitcomp/15 -> splitcomp_multiport/16
  ratechange_splitcomp/11 -> splitcomp_multiport/12
  ratechange_splitcomp/1 -> splitcomp_multiport/2
  ratechange_splitcomp/5 -> splitcomp_multiport/6
  ratechange_splitcomp/16 -> splitcomp_multiport/17
  ratechange_splitcomp/12 -> splitcomp_multiport/13
  ratechange_splitcomp/4 -> splitcomp_multiport/5
  ratechange_splitcomp/13 -> splitcomp_multiport/14
  ratechange_splitcomp/7 -> splitcomp_multiport/8
  ratechange_splitcomp/3 -> splitcomp_multiport/4
  ratechange_splitcomp/8 -> splitcomp_multiport/9
  ratechange_splitcomp/9 -> splitcomp_multiport/10
